simulink model "wattcredit_plug_sim"  (R2023a)
settings: Solver=FixedStepDiscrete  StartTime=0.0  StopTime=StopTime  FixedStep=Tp  RelTol=1e-3
values from neighbouring files (symbols this model uses):
  codes = scenario.codes    [wc_params.m]
  E = [zeros(1,4) ones(1,4) zeros(1,4) ones(1,4) 0 0 1 0 0 rule.iOffA]    [wc_params.m]
  f0 = 50    [wc_params.m]
  fRip = 1.8    [wc_params.m]
  Gi = 1/Rsh    (= 200)    [wc_params.m]
  IfsPk = 15    [wc_params.m]
  ledC = 220e-6    (= 0.00022)    [wc_params.m]
  ledR = 2000    [wc_params.m]
  ledRs = 20    [wc_params.m]
  motorIdle = derive(38, 0.28)    [wc_params.m]
  motorWork = derive(220, 0.80)    [wc_params.m]
  noiseI = 1e-3    (= 0.001)    [wc_params.m]
  noiseV = 0.05    [wc_params.m]
  pvec = [fs f0 NC Vnom prot.Vlo prot.Vhi prot.Imax prot.debounceFrames]    [wc_params.m]
  Rheater = Vnom^2/heaterP    (= 52.9)    [wc_params.m]
  Rrip = 1800    [wc_params.m]
  Rsh = 5e-3    (= 0.005)    [wc_params.m]
  Rspoof = Vnom^2/spoofHeaterP    [wc_params.m]
  segT = scenario.segT    [wc_params.m]
  Tp = Ts/4    [build_wattcredit_sim_f.m]    (also in wc_params.m = 3.90625e-05)
  Ts = 1/fs    (= 0.00015625)    [wc_params.m]
  VfsPk = 400    [wc_params.m]
  Vpk = Vnom*sqrt(2)    [wc_params.m]
libraries: spsSeriesRLCBranchLib x9, spsIdealSwitchLib x6, spsDiodeLib x4, spsVoltageMeasurementLib x2, spsACVoltageSourceLib x1, spspowerguiLib x1
settings Model: Creator=ruthm  LastModifiedBy=ruthm

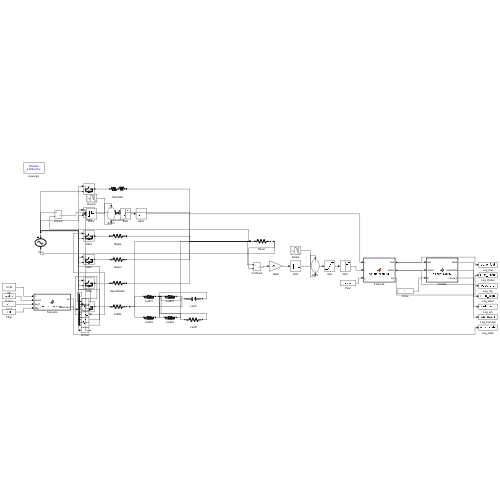
[thumbnail: Simulink's stored preview of the top-level diagram]
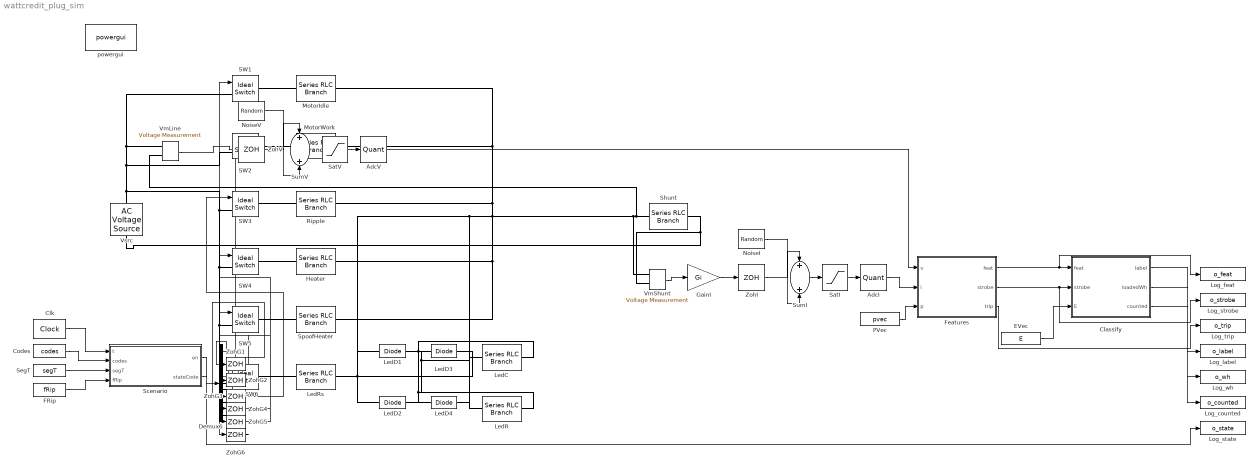
== system wattcredit_plug_sim ==
  AdcI : Quantizer  QuantizationInterval=lsbI
  AdcV : Quantizer  QuantizationInterval=lsbV
  Classify : MATLAB Function  TreatAsAtomicUnit=on
  Clk : DigitalClock  SampleTime=Ts
  Codes : Constant  Value=codes
  Demux6 : Demux  Outputs=6
  EVec : Constant  Value=E
  FRip : Constant  Value=fRip
  Features : MATLAB Function  TreatAsAtomicUnit=on
  GainI : Gain  Gain=Gi
  Heater : spsSeriesRLCBranchLib/Series RLC Branch  LConnTagsString=__new0  RConnTagsString=__new0  BranchType=R  Resistance=Rheater  Inductance=1e-3  SetiL0=off  InitialCurrent=0  Capacitance=1e-6  Setx0=off  InitialVoltage=0  Measurements=None
  LedC : spsSeriesRLCBranchLib/Series RLC Branch  LConnTagsString=__new0  RConnTagsString=__new0  BranchType=C  Resistance=1  Inductance=1e-3  SetiL0=off  InitialCurrent=0  Capacitance=ledC  Setx0=off  InitialVoltage=0  Measurements=None
  LedD{1..4} (4 alike) : spsDiodeLib/Diode  Ron=1e-3  Lon=0  Vf=0.8  IC=0  UseSnubber=0  Rs=500  Cs=250e-9  Measurements=off
  LedR : spsSeriesRLCBranchLib/Series RLC Branch  LConnTagsString=__new0  RConnTagsString=__new0  BranchType=R  Resistance=ledR  Inductance=1e-3  SetiL0=off  InitialCurrent=0  Capacitance=1e-6  Setx0=off  InitialVoltage=0  Measurements=None
  LedRs : spsSeriesRLCBranchLib/Series RLC Branch  LConnTagsString=__new0  RConnTagsString=__new0  BranchType=R  Resistance=ledRs  Inductance=1e-3  SetiL0=off  InitialCurrent=0  Capacitance=1e-6  Setx0=off  InitialVoltage=0  Measurements=None
  Log_counted : ToWorkspace  VariableName=o_counted  SampleTime=-1
  Log_feat : ToWorkspace  VariableName=o_feat  SampleTime=-1
  Log_label : ToWorkspace  VariableName=o_label  SampleTime=-1
  Log_state : ToWorkspace  VariableName=o_state  SampleTime=-1
  Log_strobe : ToWorkspace  VariableName=o_strobe  SampleTime=-1
  Log_trip : ToWorkspace  VariableName=o_trip  SampleTime=-1
  Log_wh : ToWorkspace  VariableName=o_wh  SampleTime=-1
  MotorIdle : spsSeriesRLCBranchLib/Series RLC Branch  LConnTagsString=__new0  RConnTagsString=__new0  BranchType=RL  Resistance=motorIdle.R  Inductance=motorIdle.L  SetiL0=off  InitialCurrent=0  Capacitance=1e-6  Setx0=off  InitialVoltage=0  Measurements=None
  MotorWork : spsSeriesRLCBranchLib/Series RLC Branch  LConnTagsString=__new0  RConnTagsString=__new0  BranchType=RL  Resistance=motorWork.R  Inductance=motorWork.L  SetiL0=off  InitialCurrent=0  Capacitance=1e-6  Setx0=off  InitialVoltage=0  Measurements=None
  NoiseI : RandomNumber  Variance=noiseI^2  Seed=12  SampleTime=Ts
  NoiseV : RandomNumber  Variance=noiseV^2  Seed=11  SampleTime=Ts
  PVec : Constant  Value=pvec
  Ripple : spsSeriesRLCBranchLib/Series RLC Branch  LConnTagsString=__new0  RConnTagsString=__new0  BranchType=R  Resistance=Rrip  Inductance=1e-3  SetiL0=off  InitialCurrent=0  Capacitance=1e-6  Setx0=off  InitialVoltage=0  Measurements=None
  SW{1..6} (6 alike) : spsIdealSwitchLib/Ideal Switch  Ron=1e-3  Lon=0  IC=0  Rs=1e6  Cs=inf  Measurements=off
  SatI : Saturate  UpperLimit=IfsPk  LowerLimit=-IfsPk
  SatV : Saturate  UpperLimit=VfsPk  LowerLimit=-VfsPk
  Scenario : MATLAB Function  TreatAsAtomicUnit=on
  SegT : Constant  Value=segT
  Shunt : spsSeriesRLCBranchLib/Series RLC Branch  LConnTagsString=__new0  RConnTagsString=__new0  BranchType=R  Resistance=Rsh  Inductance=1e-3  SetiL0=off  InitialCurrent=0  Capacitance=1e-6  Setx0=off  InitialVoltage=0  Measurements=None
  SpoofHeater : spsSeriesRLCBranchLib/Series RLC Branch  LConnTagsString=__new0  RConnTagsString=__new0  BranchType=R  Resistance=Rspoof  Inductance=1e-3  SetiL0=off  InitialCurrent=0  Capacitance=1e-6  Setx0=off  InitialVoltage=0  Measurements=None
  SumI : Sum
  SumV : Sum
  VmLine : spsVoltageMeasurementLib/Voltage Measurement  PhasorSimulation=off  OutputType=Complex  PSBequivalent=0
  VmShunt : spsVoltageMeasurementLib/Voltage Measurement  PhasorSimulation=off  OutputType=Complex  PSBequivalent=0
  Vsrc : spsACVoltageSourceLib/AC Voltage Source  Amplitude=Vpk  Phase=0  Frequency=f0  SampleTime=0  Measurements=None  BusType=swing  Pref=10e3  Qref=0  Qmin=-inf  Qmax=+inf
  ZohG{1..6} (6 alike) : ZeroOrderHold  SampleTime=Tp
  ZohI : ZeroOrderHold  SampleTime=Ts
  ZohV : ZeroOrderHold  SampleTime=Ts
  powergui : spspowerguiLib/powergui  Priority=1  SimulationMode=Discrete  SampleTime=Tp  frequency=60  Iterations=50  frequencyindice=50  Pbase=100e6  ErrMax=1e-4  UnitsV=kV  UnitsW=MW  buscounter=0  FunctionMessages=off  echomessages=off  EnableUseOfTLC=off  CurrentSourceSwitches=off  DisableSnubberDevices=off  DisableRonSwitches=off  DisableVfSwitches=off  DisplayEquations=off  AutomaticDiscreteSolvers=off  SolverType=Tustin/Backward Euler (TBE)  Interpol=off  ExternalGateDelay=off  methode=off  Ts=100  x0status=blocks  SPID=on  SwTol=0  HookPort=off  NonlinearTolerance=1e-4  nMaxIteration=100  ContinueOnMaxIteration=off  RestoreLinks=warning  ResistiveCurrentMeasurement=off  Frange=[0:2:500]  Ylog=off  Xlog=on  ShowGrid=off  save=off  variable=ZData  structure=0  ZoomFFT=off  StartTime=0.0  cycles=1  DisplayStyle=1  fundamental=60  FreqAxis=off  MaxFrequency=1000  frequencyindicesteady=1  RmsSteady=1  display=off
  wires:
  VmLine/1 -> ZohV/1
  ZohV/1 -> SumV/1
  NoiseV/1 -> SumV/2
  SumV/1 -> SatV/1
  SatV/1 -> AdcV/1
  VmShunt/1 -> GainI/1
  GainI/1 -> ZohI/1
  ZohI/1 -> SumI/1
  NoiseI/1 -> SumI/2
  SumI/1 -> SatI/1
  SatI/1 -> AdcI/1
  AdcV/1 -> Features/1(v)
  AdcI/1 -> Features/2(i)
  PVec/1 -> Features/3(p)
  Features/1(feat) -> Classify/1(feat), Log_feat/1
  Features/2(strobe) -> Classify/2(strobe), Log_strobe/1
  EVec/1 -> Classify/3(E)
  Clk/1 -> Scenario/1(t)
  Codes/1 -> Scenario/2(codes)
  SegT/1 -> Scenario/3(segT)
  FRip/1 -> Scenario/4(fRip)
  Scenario/1(en) -> Demux6/1
  Demux6/1 -> ZohG1/1
  ZohG1/1 -> SW1/1
  Demux6/2 -> ZohG2/1
  ZohG2/1 -> SW2/1
  Demux6/3 -> ZohG3/1
  ZohG3/1 -> SW3/1
  Demux6/4 -> ZohG4/1
  ZohG4/1 -> SW4/1
  Demux6/5 -> ZohG5/1
  ZohG5/1 -> SW5/1
  Demux6/6 -> ZohG6/1
  ZohG6/1 -> SW6/1
  Features/3(trip) -> Log_trip/1
  Classify/1(label) -> Log_label/1
  Classify/2(loadedWh) -> Log_wh/1
  Classify/3(counted) -> Log_counted/1
  Scenario/2(stateCode) -> Log_state/1
  connections:
  SW1/LConn1 -- Vsrc/RConn1 -- SW5/LConn1 -- SW6/LConn1 -- SW4/LConn1 -- SW3/LConn1 -- SW2/LConn1 -- VmLine/LConn1
  SW1/RConn1 -- MotorIdle/LConn1
  SW2/RConn1 -- MotorWork/LConn1
  SW3/RConn1 -- Ripple/LConn1
  SW4/RConn1 -- Heater/LConn1
  SW5/RConn1 -- SpoofHeater/LConn1
  SW6/RConn1 -- LedRs/LConn1
  MotorIdle/RConn1 -- SpoofHeater/RConn1 -- Heater/RConn1 -- LedD4/RConn1 -- LedD2/LConn1 -- Shunt/LConn1 -- VmLine/LConn2 -- VmShunt/LConn1 -- Ripple/RConn1 -- MotorWork/RConn1
  Vsrc/LConn1 -- Shunt/RConn1 -- VmShunt/LConn2
  LedD1/LConn1 -- LedRs/RConn1 -- LedD3/RConn1
  LedD2/RConn1 -- LedD1/RConn1 -- LedC/LConn1 -- LedR/LConn1
  LedD4/LConn1 -- LedD3/LConn1 -- LedC/RConn1 -- LedR/RConn1

== matlab function wattcredit_plug_sim/Classify ==
  data: feat input; label output; strobe input; E input; loadedWh output; counted output
function [label, loadedWh, counted] = wc_fcn_classify(feat, strobe, E)
%WC_FCN_CLASSIFY  Frame-rate evidence rule (paste into a MATLAB Function block).
%  feat    : [pf h3 h5 ripple pnorm irms vrms]
%  strobe  : 1 when feat holds a new 1 s frame
%  E       : enrolment vector, 22 elements
%            E(1:4) muIdle, E(5:8) sdIdle, E(9:12) muWork, E(13:16) sdWork,
%            E(17) pnIdle, E(18) pnWork, E(19) tau, E(20) pGate, E(21) ripGate, E(22) iOff
%  label   : 0 OFF, 1 IDLE, 2 WORK, 3 OTHER (held between frames)
%  counted : 1 on the frame in which a WORK frame was credited
%  loadedWh: cumulative energy above the idle baseline, credited only on WORK frames
persistent lab wh
if isempty(lab), lab = 0; wh = 0; end
f  = feat(:);                                     % force column vectors: row/column mix-ups broadcast silently
Ev = E(:);
counted = 0;
if strobe
    x  = f(1:4);
    dI = sqrt(mean(((x - Ev(1:4)) ./ Ev(5:8)).^2));
    dW = sqrt(mean(((x - Ev(9:12)) ./ Ev(13:16)).^2));
    if f(6) < Ev(22)
        lab = 0;                                  % OFF
    elseif min(dI, dW) > Ev(19)
        lab = 3;                                  % not the enrolled signature: never counted
    elseif dW < dI && f(5) >= Ev(20) && f(4) >= Ev(21)
        lab = 2;                                  % authentic loaded work
        wh = wh + max(f(5) - Ev(17), 0)/3600;   % 1 s frame
        counted = 1;
    else
        lab = 1;                                  % enrolled machine, idle
    end
end
label = lab;
loadedWh = wh;
end

== matlab function wattcredit_plug_sim/Features ==
  data: v input; feat output; i input; p input; strobe output; trip output
function [feat, strobe, trip] = wc_fcn_features(v, i, p)
%WC_FCN_FEATURES  Sample-rate feature extractor (paste into a MATLAB Function block).
%  v, i   : ADC-processed voltage (V) and current (A), one sample per Ts
%  p      : [fs f0 NC Vnom Vlo Vhi Imax debounceFrames]
%  feat   : [pf h3 h5 ripple pnorm irms vrms], valid when strobe = 1 (once per 1 s frame)
%  trip   : protection flag, raised after debounceFrames bad frames. Detect-only: nothing is switched.
%
%  Cycle-synchronous: one cycle = fs/f0 samples, one frame = NC cycles. Harmonic k is correlated
%  against sin/cos of k*f0 over the whole frame (equals the frame FFT bin k*NC).
spc = round(p(1)/p(2));  NC = round(p(3));  N = spc*NC;
persistent n cyc sv2 si2 svi c1 s1 c3 s3 c5 s5 cs2 cycR badCnt tripState lastFeat
if isempty(n)
    n = 0; cyc = 0; sv2 = 0; si2 = 0; svi = 0;
    c1 = 0; s1 = 0; c3 = 0; s3 = 0; c5 = 0; s5 = 0; cs2 = 0;
    cycR = zeros(1, 200);  badCnt = 0; tripState = 0; lastFeat = zeros(1, 7);
end
th = 2*pi*mod(n, spc)/spc;
sv2 = sv2 + v*v;   si2 = si2 + i*i;   svi = svi + v*i;
cs2 = cs2 + i*i;                                  % current energy inside the present cycle
c1 = c1 + i*cos(th);    s1 = s1 + i*sin(th);
c3 = c3 + i*cos(3*th);  s3 = s3 + i*sin(3*th);
c5 = c5 + i*cos(5*th);  s5 = s5 + i*sin(5*th);
n = n + 1;
strobe = 0;
if mod(n, spc) == 0                               % end of a cycle
    cyc = cyc + 1;
    cycR(cyc) = sqrt(cs2/spc);   cs2 = 0;
end
if n >= N                                         % end of a frame
    vrms = sqrt(sv2/N);   irms = sqrt(si2/N);   P = svi/N;
    if vrms*irms > 1e-9, pf = P/(vrms*irms); else, pf = 0; end
    a1 = 2/N*sqrt(c1^2 + s1^2);  a3 = 2/N*sqrt(c3^2 + s3^2);  a5 = 2/N*sqrt(c5^2 + s5^2);
    if a1 > 1e-4, h3 = a3/a1; h5 = a5/a1; else, h3 = 0; h5 = 0; end
    r = cycR(1:cyc);   mr = mean(r);
    if mr > 1e-4, rip = sqrt(mean((r - mr).^2))/mr; else, rip = 0; end
    pn = P*(p(4)/max(vrms, 1))^2;
    lastFeat = [pf h3 h5 rip pn irms vrms];
    bad = (vrms < p(5)) || (vrms > p(6)) || (irms > p(7));
    if bad, badCnt = badCnt + 1; else, badCnt = 0; tripState = 0; end
    if badCnt >= p(8), tripState = 1; end
    strobe = 1;
    n = 0; cyc = 0; sv2 = 0; si2 = 0; svi = 0; c1 = 0; s1 = 0; c3 = 0; s3 = 0; c5 = 0; s5 = 0; cs2 = 0;
end
feat = lastFeat(:);                                % 7x1 column: a 1-D vector signal in Simulink
trip = tripState;
end

== matlab function wattcredit_plug_sim/Scenario ==
  data: t input; en output; codes input; segT input; fRip input; stateCode output
function [en, stateCode] = wc_fcn_scenario(t, codes, segT, fRip)
%WC_FCN_SCENARIO  Turns a list of state codes into breaker enables (paste into a MATLAB Function block).
%  codes : 0 OFF, 1 IDLE, 2 WORK, 3 HEATER, 4 LED, 5 SPOOF (idle motor + steady heater)
%  en    : [idleMotor workMotor ripple heater spoofHeater led], 1 = breaker closed
idx = min(floor(t/segT) + 1, numel(codes));
c = codes(idx);
tog = double(mod(floor(t*fRip*2), 2) == 0);
en = [double(c == 1 || c == 5), double(c == 2), double(c == 2)*tog, double(c == 3), double(c == 5), double(c == 4)]';   % column, so Simulink sees a 1-D vector for the Demux
stateCode = c;
end
